simulink model "planta_rots"  (R2025b)
settings: Solver=VariableStepAuto  StartTime=0.0  StopTime=1000  RelTol=1e-3
values from neighbouring files (symbols this model uses):
  ah_max = 0.75    [init_plant_parameters.m]
  at_max = 0.80    (= 0.8)    [init_plant_parameters.m]
  bcx = 1.0e6    (= 1000000)    [init_plant_parameters.m]
  bcy = 10.0e6    (= 10000000)    [init_plant_parameters.m]
  bh_eq = bhm+bhd/ih^2    (= 18.0165289256)    [init_plant_parameters.m]
  bhb = 100e6    (= 100000000)    [init_plant_parameters.m]
  bhEb = 2.2e9    (= 2200000000)    [init_plant_parameters.m]
  bhwu = 150    [init_plant_parameters.m]
  bt = 90.0    (= 90)    [init_plant_parameters.m]
  bt_eq = btm+btd/it^2    (= 6.002)    [init_plant_parameters.m]
  btb = 5.0e6    (= 5000000)    [init_plant_parameters.m]
  btw = 3.0e3    (= 3000)    [init_plant_parameters.m]
  counter_limit = timeout/(Ts0*1000)    (= 1500)    [init_plant_parameters.m]
  envolvent = [ones(1,N_xt)]*38    [init_plant_parameters.m]
  g = 9.80665    [init_plant_parameters.m]
  Hc = 2.59    [init_plant_parameters.m]
  ih = 22.0    (= 22)    [init_plant_parameters.m]
  it = 30.0    (= 30)    [init_plant_parameters.m]
  Jh_eq = Jhm_hb+Jhd_hEb/ih^2    (= 37.8512396694)    [init_plant_parameters.m]
  Jt_eq = Jtm_tb+Jtd/it^2    (= 8.33333333333)    [init_plant_parameters.m]
  k_i_c = abs(polos_obs_c)^3    [init_plant_parameters.m]
  k_i_h = abs(polos_obs_h)^3    [init_plant_parameters.m]
  k_omega_c = 3 * abs(polos_obs_c)^2    [init_plant_parameters.m]
  k_omega_h = 3 * abs(polos_obs_h)^2-k_tita_h*bh_eq/Jh_eq    [init_plant_parameters.m]
  k_tita_c = 3 * abs(polos_obs_c)    [init_plant_parameters.m]
  k_tita_h = 3 * abs(polos_obs_h)-bh_eq/Jh_eq    [init_plant_parameters.m]
  Kcy = 1.8e9    (= 1800000000)    [init_plant_parameters.m]
  khwu = 236e6    (= 236000000)    [init_plant_parameters.m]
  Ki_c = (wn_t^2*Mt)/Kf    (= 320)    [init_plant_parameters.m]
  Ki_i = (wn_h^2)*Jh_eq    (= 2422.47933884)    [init_plant_parameters.m]
  Kp_c = (2*zitta_t*wn_t*Mt)/Kf    (= 1120)    [init_plant_parameters.m]
  Kp_i = 2*zitta_h*wn_h*Jh_eq    (= 1211.23966942)    [init_plant_parameters.m]
  Ktw = 480e3    (= 480000)    [init_plant_parameters.m]
  Lh0 = 110    [init_plant_parameters.m]
  lh_0 = Yt0-yh_0    (= 7)    [init_plant_parameters.m]
  Mc_max = 50000    [init_plant_parameters.m]
  Mc_min = 2000    [init_plant_parameters.m]
  Ms = 15000    [init_plant_parameters.m]
  Mt = 30000    [init_plant_parameters.m]
  P_nom = 956150    [init_plant_parameters.m]
  periodo_pulsos = 100    [init_plant_parameters.m]
  rhd = 0.75    [init_plant_parameters.m]
  rtd = 0.50    (= 0.5)    [init_plant_parameters.m]
  tau_hm = Ts2    (= 0.001)    [init_plant_parameters.m]
  tau_tm = Ts2    (= 0.001)    [init_plant_parameters.m]
  Thb_Max = 50e3    (= 50000)    [init_plant_parameters.m]
  ThEb_Max = 1.1e6    (= 1100000)    [init_plant_parameters.m]
  Thm_0 = 0    [init_plant_parameters.m]
  Thm_Max = 20e3    (= 20000)    [init_plant_parameters.m]
  titahm_0 = yl_0/(rhd/(2*ih))    (= 2228.19975108)    [init_plant_parameters.m]
  titatm_0 = xtd_0/(rtd/it)    (= 300)    [init_plant_parameters.m]
  Ts0 = 0.02    [init_plant_parameters.m]
  Ts1 = 0.02    [init_plant_parameters.m]
  Ts2 = 0.001    [init_plant_parameters.m]
  Ttb_Max = 5.0e3    (= 5000)    [init_plant_parameters.m]
  Ttm_0 = 0    [init_plant_parameters.m]
  Ttm_Max = 4.0e3    (= 4000)    [init_plant_parameters.m]
  vh_0 = 0    [init_plant_parameters.m]
  vh_max = 3    [init_plant_parameters.m]
  vh_nom = 1.5    [init_plant_parameters.m]
  vt_0 = 0    [init_plant_parameters.m]
  vt_max = 4.0    (= 4)    [init_plant_parameters.m]
  Wc = 2.44    [init_plant_parameters.m]
  x_LIDAR = 3    [init_plant_parameters.m]
  xl_0 = 5    [init_plant_parameters.m]
  xt_0 = 5    [init_plant_parameters.m]
  xt_max = 50.0    (= 50)    [init_plant_parameters.m]
  xt_min = -30.0    (= -30)    [init_plant_parameters.m]
  xtd_0 = xt_0    (= 5)    [init_plant_parameters.m]
  yc0_vec_inicial = [ 0, 0, 1, 0, 0, 1, 0, 0, 0, 0, 0, 0, alt_borde,                   3, 5, 6, 3, 5, 6, 6, 4, 1, 1, -4, -5, -2, -1, 2, 6, 4, 2, 5,                   alt_borde] * Hc    [init_plant_parameters.m]
  yh_max = 40    [init_plant_parameters.m]
  yh_min = -20    [init_plant_parameters.m]
  yl_0 = Yt0 - l_0    (= 37.9806775752)    [init_plant_parameters.m]
  Yt0 = 45.0    (= 45)    [init_plant_parameters.m]
  zitta = 0.5    [init_plant_parameters.m]
undefined symbols (not defined in the file or in its folder): DiscIntNeverNeededParam
libraries: dspnetwork x2, sl3dlib x1, simulink_extras x1, hostiolib x1
(part 2 of 2)

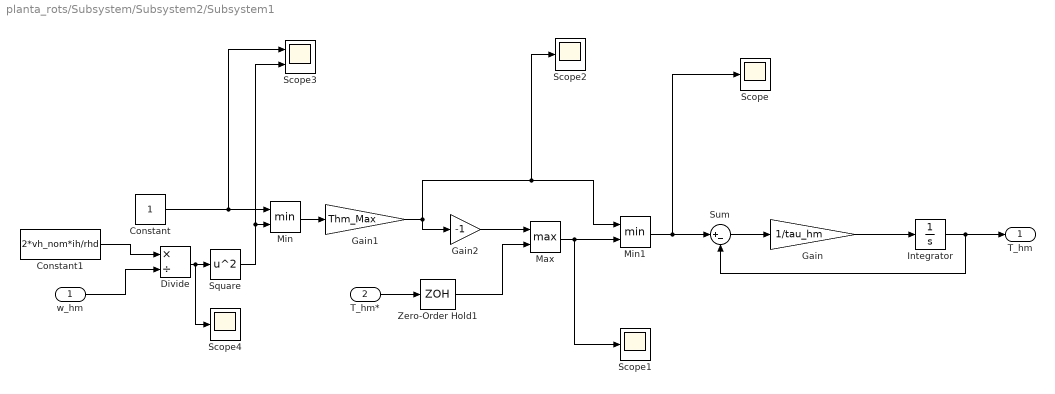
== system planta_rots/Subsystem/Subsystem2/Subsystem1 ==
  w_hm : Inport
  T_hm* : Inport  Port=2
  Constant : Constant
  Constant1 : Constant  Value=2*vh_nom*ih/rhd
  Divide : Product  Inputs=*/
  Gain : Gain  Gain=1/tau_hm
  Gain1 : Gain  Gain=Thm_Max
  Gain2 : Gain  Gain=-1
  Integrator : Integrator
  Max : MinMax  Function=max  Inputs=2
  Min : MinMax  Inputs=2
  Min1 : MinMax  Inputs=2
  Scope{,1..2,4} (4 alike) : Scope
      Scope settings: ActiveDisplayYMinimum=-2500  ActiveDisplayYMaximum=22500  DataLoggingVariableName=ScopeData3
      Scope1 settings: ActiveDisplayYMinimum=-2500  ActiveDisplayYMaximum=22500  DataLoggingVariableName=ScopeData4
      Scope2 settings: ActiveDisplayYMinimum=481.45655  ActiveDisplayYMaximum=22168.72705  DataLoggingVariableName=ScopeData5
      Scope4 settings: ActiveDisplayYMinimum=-0.06596  ActiveDisplayYMaximum=-0.00953  DataLoggingVariableName=ScopeData7
  Scope3 : Scope  NumInputPorts=2
      settings: ActiveDisplayYMinimum=-9.1717430786370772E+28  ActiveDisplayYMaximum=8.25456877077337E+29  DataLoggingVariableName=ScopeData6
  Square : Math  Operator=square
  Sum : Sum  Inputs=|+-
  Zero-Order Hold1 : ZeroOrderHold  SampleTime=tau_hm
  T_hm : Outport
  wires:
  Sum/1 -> Gain/1
  Gain/1 -> Integrator/1
  Integrator/1 -> Sum/2, T_hm/1
  Constant/1 -> Scope3/1, Min/1
  w_hm/1 -> Divide/2
  Constant1/1 -> Divide/1
  Divide/1 -> Scope4/1, Square/1
  Square/1 -> Scope3/2, Min/2
  Min/1 -> Gain1/1
  Gain1/1 -> Scope2/1, Min1/1, Gain2/1
  T_hm*/1 -> Zero-Order Hold1/1
  Gain2/1 -> Max/1
  Max/1 -> Scope1/1, Min1/2
  Min1/1 -> Scope/1, Sum/1
  Zero-Order Hold1/1 -> Max/2

== system planta_rots/Subsystem/accionamiento izaje/brake izaje ==
  w_hm : Inport
  BRK_h : Inport  Port=2
  Constant : Constant  Value=0
  Gain : Gain  Gain=bhb
  Gain1 : Gain  Gain=-Thb_Max
  Switch : Switch  Criteria=u2 > Threshold  SaturateOnIntegerOverflow=off  InputSameDT=off
  Tanh : Trigonometry  Operator=tanh
  T_hb : Outport
  wires:
  Switch/1 -> T_hb/1
  Constant/1 -> Switch/1
  BRK_h/1 -> Switch/2
  w_hm/1 -> Gain/1
  Gain/1 -> Tanh/1
  Tanh/1 -> Gain1/1
  Gain1/1 -> Switch/3

== system planta_rots/Subsystem/accionamiento izaje/brake izaje emergencia ==
  w_hd : Inport
  BRK_hE : Inport  Port=2
  Constant : Constant  Value=0
  Gain : Gain  Gain=bhEb
  Gain1 : Gain  Gain=-ThEb_Max
  Switch : Switch  Criteria=u2 > Threshold  SaturateOnIntegerOverflow=off  InputSameDT=off
  Tanh : Trigonometry  Operator=tanh
  T_hEb : Outport
  wires:
  Tanh/1 -> Gain1/1
  Gain/1 -> Tanh/1
  Constant/1 -> Switch/1
  w_hd/1 -> Gain/1
  Switch/1 -> T_hEb/1
  BRK_hE/1 -> Switch/2
  Gain1/1 -> Switch/3

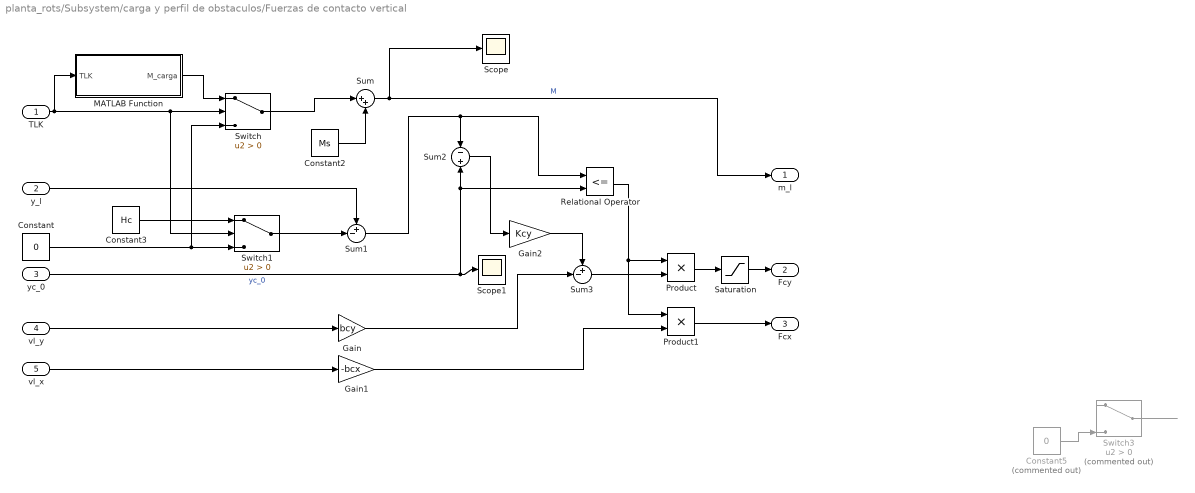
== system planta_rots/Subsystem/carga y perfil de obstaculos/Fuerzas de contacto vertical ==
  TLK : Inport
  y_l : Inport  Port=2
  yc_0 : Inport  Port=3
  vl_y : Inport  Port=4
  vl_x : Inport  Port=5
  Constant : Constant  Value=0
  Constant2 : Constant  Value=Ms
  Constant3 : Constant  Value=Hc
  Constant5 : Constant  Commented=on  Value=0
  Gain : Gain  Gain=bcy
  Gain1 : Gain  Gain=-bcx
  Gain2 : Gain  Gain=Kcy
  MATLAB Function : MATLAB Function  TreatAsAtomicUnit=on
  Product : Product
  Product1 : Product
  Relational Operator : RelationalOperator  Operator=<=  OutDataTypeStr=boolean  RndMeth=Simplest  InputSameDT=off
  Saturation : Saturate  UpperLimit=inf  LowerLimit=0
  Scope : Scope
      settings: ActiveDisplayYMinimum=-30040.049311756404  ActiveDisplayYMaximum=65258.780060315854  DataLoggingVariableName=ScopeData31
  Scope1 : Scope
      settings: ActiveDisplayYMinimum=12.776564460216019  ActiveDisplayYMaximum=15.5369149188378  DataLoggingVariableName=ScopeData32
  Sum : Sum  Inputs=|++
  Sum1 : Sum  Inputs=+-|
  Sum2 : Sum  Inputs=-|+
  Sum3 : Sum  Inputs=+-|
  Switch : Switch  Criteria=u2 > Threshold  SaturateOnIntegerOverflow=off  InputSameDT=off
  Switch1 : Switch  Criteria=u2 > Threshold  SaturateOnIntegerOverflow=off  InputSameDT=off
  Switch3 : Switch  Commented=on  Criteria=u2 > Threshold  SaturateOnIntegerOverflow=off  InputSameDT=off
  m_l : Outport
  Fcy : Outport  Port=2
  Fcx : Outport  Port=3
  wires:
  MATLAB Function/1(M_carga) -> Switch/1
  TLK/1 -> MATLAB Function/1(TLK), Switch1/2, Switch/2
  Constant/1 -> Switch1/3, Switch/3
  Constant3/1 -> Switch1/1
  Switch/1 -> Sum/1
  Sum/1 -> Scope/1, m_l/1  "M"
  Constant2/1 -> Sum/2
  Switch1/1 -> Sum1/2
  y_l/1 -> Sum1/1
  Sum1/1 -> Relational Operator/1, Sum2/1
  yc_0/1 -> Scope1/1, Sum2/2, Relational Operator/2  "yc_0"
  Sum2/1 -> Gain2/1
  Gain2/1 -> Sum3/1
  Relational Operator/1 -> Product1/1, Product/1
  Product1/1 -> Fcx/1
  Gain/1 -> Sum3/2
  vl_y/1 -> Gain/1
  vl_x/1 -> Gain1/1
  Gain1/1 -> Product1/2
  Sum3/1 -> Product/2
  Constant5/1 -> Switch3/3
  Switch3/1 -> ?
  ? -> Switch3/1, Switch3/2
  Product/1 -> Saturation/1
  Saturation/1 -> Fcy/1

== matlab function planta_rots/Subsystem/carga y perfil de obstaculos/MATLAB Function ==
  data: y0_array input; yc0_xt output; index input
function yc0_xt= calcula_y0(y0_array,index)
index = floor(index)+1;
index = min(max(index,1),33);
yc0_xt = y0_array(index);

== stateflow chart planta_rots/Nivel 0 ==
  state Muerto
    entry:
    BRK_hE_N0 = 0; BRK_t_N0 = 0;
  state Name
    state ESTADOS_SEGURIDAD [parallel]
      entry:
      vh_lim = vh_max;
      settings: executionOrder=1
      state SISTEMA_OK
        entry:
        BRK_hE_N0 = 1; BRK_t_N0 = 1;
        FALLA_MAN = 0; FALLA_WD = 0;
        FALLA_IZAJE_SUP = 0; FALLA_IZAJE_INF = 0;
        FALLA_IZAJE_SV = 0;
        FALLA_CARRO_DER = 0; FALLA_CARRO_IZQ = 0;
        during:
        vh_lim = min(vh_max,...
        max(vh_nom, (P_nom / ((m_cont + Ms) * g))));
      state MODO_RECUPERACION
        entry:
        BRK_hE_N0 = 1; BRK_t_N0 = 1;
        FALLA_MAN = 0;
        FALLA_IZAJE_SV = 0;
      state EMERGENCIA_MANUAL
        entry:
        BRK_hE_N0 = 0; BRK_t_N0 = 0;
        FALLA_MAN = 1;
      state EMERGENCIA_IZAJE_INF
        entry:
        BRK_hE_N0 = 0; BRK_t_N0 = 1;
        FALLA_IZAJE_INF = 1;
      state EMERGENCIA_IZAJE_SUP
        entry:
        BRK_hE_N0 = 0; BRK_t_N0 = 1;
        FALLA_IZAJE_SUP = 1;
      state EMERGENCIA_CARRO_SV
        entry:
        BRK_hE_N0 = 1; BRK_t_N0 = 0;
        FALLA_CARRO_SV = 1;
      state EMERGENCIA_CARRO_DER
        entry:
        BRK_hE_N0 = 1; BRK_t_N0 = 0;
        FALLA_CARRO_DER = 1;
      state EMERGENCIA_CARRO_IZQ
        entry:
        BRK_hE_N0 = 1; BRK_t_N0 = 0;
        FALLA_CARRO_IZQ = 1;
      state EMERGENCIA_IZAJE_SV
        entry:
        BRK_hE_N0 = 0; BRK_t_N0 = 1;
        FALLA_IZAJE_SV = 1;
      (default) -> SISTEMA_OK
      MODO_RECUPERACION -> SISTEMA_OK : [recup_ok == 1]
      (junction 76) -> MODO_RECUPERACION : [BTN_Reset]
      SISTEMA_OK -> (junction 55) [order 3]
      SISTEMA_OK -> (junction 48) [order 2]
      SISTEMA_OK -> EMERGENCIA_MANUAL [order 1] : [BTN_Emerg]
      EMERGENCIA_MANUAL -> (junction 76)
      (junction 78) -> (junction 76)
      (junction 55) -> EMERGENCIA_IZAJE_SV [order 3] : [abs(vh_obs) > (1.15 * vh_lim)]
      (junction 55) -> EMERGENCIA_CARRO_SV [order 4] : [abs(vt_obs) > (1.15 * vt_max)]
      (junction 48) -> EMERGENCIA_CARRO_DER [order 2] : [FCE_der == 1]
      (junction 48) -> EMERGENCIA_CARRO_IZQ [order 1] : [FCE_izq == 1]
      (junction 55) -> EMERGENCIA_IZAJE_INF [order 2] : [FCE_inf == 1]
      (junction 55) -> EMERGENCIA_IZAJE_SUP [order 1] : [FCE_sup == 1]
      EMERGENCIA_CARRO_DER -> (junction 84)
      EMERGENCIA_CARRO_IZQ -> (junction 84)
      EMERGENCIA_IZAJE_INF -> (junction 84)
      EMERGENCIA_IZAJE_SUP -> (junction 78)
      EMERGENCIA_CARRO_SV -> (junction 78)
      EMERGENCIA_IZAJE_SV -> (junction 78)
      (junction 84) -> (junction 78)
    state WATCHDOG [parallel]
      settings: executionOrder=2
      state HEARTBEAT_DOWN
        entry:
        WD_counter = 0;
        during:
        WD_counter = WD_counter + 1;
      state DETECCION_FALLO
        entry:
        FALLA_WD = 1;
      state HEARTBEAT_UP
        entry:
        WD_counter = 0;
        during:
        WD_counter = WD_counter + 1;
      (default) -> HEARTBEAT_DOWN
      HEARTBEAT_DOWN -> DETECCION_FALLO [order 2] : [WD_counter >= counter_limit]
      HEARTBEAT_UP -> HEARTBEAT_DOWN [order 1] : [heartbeat==0]
      HEARTBEAT_DOWN -> HEARTBEAT_UP [order 1] : [heartbeat==1]
      DETECCION_FALLO -> HEARTBEAT_DOWN : [FALLA_WD==0]
      HEARTBEAT_UP -> DETECCION_FALLO [order 2] : [WD_counter >= counter_limit]
  (default) -> Muerto
  Muerto -> Name : [modo_muerto==0]
  Name -> Muerto : [modo_muerto==1]
  data: BTN_Emerg input; BTN_Reset input; FCE_der input; FCE_inf input; FCE_izq input; FCE_sup input; P_nom parameter; g parameter; recup_ok input; vh_max parameter; vh_nom parameter; vh_obs input; vh_lim local; BRK_hE_N0 output; BRK_t_N0 output; FALLA_CARRO_DER output; FALLA_CARRO_IZQ output; FALLA_IZAJE_INF output; FALLA_IZAJE_SUP output; FALLA_IZAJE_SV output; FALLA_MAN output; FALLA_WD output; vt_max parameter; vt_obs input; FALLA_CARRO_SV output; modo_muerto input; counter_limit parameter; heartbeat input; WD_counter local; Ms parameter; m_cont input

== stateflow chart planta_rots/Nivel 1 ==
  state Muerto
    entry:
    modo_muerto=1;
    BRK_h_N1=0;
    BRK_t_N1=0;
    modo_reposo =0;
    TLK = 0;
    exit:
    modo_muerto=0;
  state Automata
    state AUTOMATA_PRINCIPAL [parallel]
      entry:
      ya_vuelvo = 0;
      dead_zone = 0.1; % Zona muerta joystick
      %error_der = 0; error_izq = 0;
      %error_sup = 0; error_inf = 0;
      %error_otro =1;
      %modo_manual_auto = 0;
      %ya_vuelvo = 0;
      during:
      Joy_CMD_X = Joy_XY(1);
      Joy_CMD_Y = Joy_XY(2);
      settings: executionOrder=6
      state REPOSO
        entry:
        modo_reposo = 1;
        BRK_t_N1 = 0; BRK_h_N1 = 0;
        modo_manual = 0;
        modo_manual_auto =0;
        error_der = 0; error_izq = 0;
        error_sup = 0; error_inf = 0;
        error_otro =0;
        modo_error = 0;
        exit:
        modo_reposo = 0;
      state RECUPERACION
        entry:
        BRK_t_N1 = 1; BRK_h_N1 = 1;
        vel_error = 0.1;
        recuperacion = 1;
        during:
        if (abs(Joy_CMD_X) < dead_zone)
        vx_target = 0;
        else
        vx_target = Joy_CMD_X * vt_max/3;
        if (error_der == 1)
        vx_target = Joy_CMD_X * vel_error;
        if (vx_target > 0) vx_target = 0; end
        elseif (error_izq == 1)
        vx_target = Joy_CMD_X * vel_error;
        if (vx_target < 0) vx_target = 0; end
        end
        end
        if (abs(Joy_CMD_Y) < dead_zone)
        vy_target = 0;
        else
        vy_target = Joy_CMD_Y * vh_lim/3;
        if (error_sup == 1)
        vy_target = Joy_CMD_Y * vel_error;
        if (vy_target > 0) vy_target = 0; end
        elseif (error_inf == 1)
        vy_target = Joy_CMD_Y * vel_error;
        if (vy_target < 0) vy_target = 0; end
        end
        end
        exit:
        recuperacion = 0;
        %modo_error = 1;
      state ERROR_OTRO
        entry:
        BRK_t_N1 = 0; BRK_h_N1 = 0;
        recuperacion = 0;
        error_otro = 1;
        vx_target=0,vy_target=0;
        modo_error = 1;
      state ERROR_FC_sup_inf
        entry:
        BRK_t_N1 = 1; BRK_h_N1 = 0;
        vy_target = 0;
        recuperacion = 0;
        if FC_inf==1
        error_inf=1;
        elseif FC_sup==1;
        error_sup=1;
        end
        modo_error = 1;
      state MANUAL
        entry:
        %BRK_t_N1 = 1; BRK_h_N1 = 1;
        modo_manual = 1;
        during:
        if (abs(T_hm)>(m_container+Ms)*g*0.02)
        BRK_h_N1=1;
        end
        if (abs(T_tm)>(m_container+Ms)*g*0.0002)
        BRK_t_N1=1;
        end
        if (abs(Joy_CMD_X) < dead_zone)
        vx_target = 0;
        else
        vx_target = Joy_CMD_X * vt_max;
        end
        if (abs(Joy_CMD_Y) < dead_zone)
        vy_target = 0;
        else
        vy_target = Joy_CMD_Y * vh_lim;
        end
        exit:
        modo_manual = 0;
      state ERROR_FC_izq_der
        entry:
        BRK_t_N1 = 0; BRK_h_N1 = 1;
        vx_target = 0;
        recuperacion = 0;
        if FC_der==1;
        error_der=1;
        elseif FC_izq==1;
        error_izq=1;
        end
        modo_error = 1;
      state MODO_AUTO
        entry:
        if(ya_vuelvo == 1)
        BRK_t_N1 = 1; BRK_h_N1 = 1;
        else ya_vuelvo = 0;
        end
        ciclo_doble=0;
        ejec_mov_final = 0;
        exit:
        if(ya_vuelvo == 0)
        modo_auto = 0;
        modo_manual_auto = 0;
        ejec_mov = 0;
        end
        state SEL_ORIGEN
          entry:
          i_sel = 1;
          i_origen = 0;
          cont =0;
          during:
          if (Joy_CMD_X > dead_zone) && every(50, tick)
          i_sel = i_sel + 1;
          elseif (Joy_CMD_X < -dead_zone) && every(50, tick)
          i_sel = i_sel - 1;
          end
          cont= Check_Container(i_sel,yc0_vec);
          exit:
          i_origen = i_sel;
        state SEL_DESTINO
          entry:
          i_sel = i_origen;
          i_destino = 0;
          invalido = 1;
          during:
          if (Joy_CMD_X > dead_zone) && every(50, tick)
          i_sel = i_sel + 1;
          elseif (Joy_CMD_X < -dead_zone) && every(50, tick)
          i_sel = i_sel - 1;
          end
          if (i_sel == 33 || i_sel == 13 || i_sel == 1|| i_sel==i_origen)
          invalido = 1;
          else invalido = 0;
          end
          exit:
          i_destino = i_sel;
        state AUTO_INIT
          entry:
          BRK_t_N1 = 0; BRK_h_N1 = 0;
          home = 13;
          estado = 1; % Etapa de movimiento
          if (TLK == 1)
          estado = 2;
          i_origen = 0;
          end
        state SELECCION_TRAYECTORIA
          entry:
          modo_auto = 1;
          manual_ok = 0;
          i_usado = 1;
          if (estado == 1)
          i_usado = i_origen;
          elseif (estado == 2)
          i_usado = i_destino;
          elseif (estado ==3);
          i_usado = home;
          end
        state MOVIMIENTO_CURVO
          entry: ejec_mov = 1;ya_vuelvo=0;
          during:
          if (abs(T_hm)>(m_container+Ms)*g*0.02)
          BRK_h_N1=1;
          end
          if (abs(T_tm)>(m_container+Ms)*g*0.0002)
          BRK_t_N1=1;
          end
          [vx_target, vy_target, manual_ok] = Planificador_Trayectoria_Vel(xt_enc,...
          yh_enc, vt_obs, vh_obs, i_usado, envolvente, TLK, theta_l, vh_lim);
          if (abs(Joy_XY(1)) > dead_zone || abs(Joy_XY(2)) > dead_zone)
          ya_vuelvo = 1
          end
          if (BTN_Auto ==1)
          ciclo_doble=1;
          end
          exit: ejec_mov = 0;
        state MOVIMIENTO_CURVO_FINAL
          entry: ejec_mov_final = 1;ya_vuelvo=0;
          during:
          if (abs(T_hm)>(m_container+Ms)*g*0.02)
          BRK_h_N1=1;
          end
          if (abs(T_tm)>(m_container+Ms)*g*0.0002)
          BRK_t_N1=1;
          end
          [vx_target, vy_target, manual_ok] = Planificador_Trayectoria_Vel(xt_enc,...
          yh_enc, vt_obs, vh_obs, i_usado, envolvent, TLK, theta_l, vh_lim);
          if (abs(Joy_XY(1)) > dead_zone || abs(Joy_XY(2)) > dead_zone)
          ya_vuelvo = 1
          end
          exit: ejec_mov_final = 0;
        state MODO_MANUAL_SIMPLE
          entry:
          modo_auto = 0;
          modo_manual_auto = 1;
          during:
          if (abs(T_hm)>(m_container+Ms)*g*0.02)
          BRK_h_N1=1;
          end
          if (abs(T_tm)>(m_container+Ms)*g*0.0002)
          BRK_t_N1=1;
          end
          if (abs(Joy_CMD_X) < dead_zone)
          vx_target = 0;
          else
          vx_target = Joy_CMD_X * 0.05;
          end
          if (abs(Joy_CMD_Y) < dead_zone)
          vy_target = 0;
          else
          vy_target = Joy_CMD_Y * vh_lim;
          end
          exit:
          estado = estado + 1;
          modo_manual_auto = 0;
        (default) -> (junction 347)
        (junction 347) -> MOVIMIENTO_CURVO [order 1] : [ya_vuelvo == 1]
        (junction 347) -> AUTO_INIT [order 2]
        SEL_ORIGEN -> SEL_DESTINO : [BTN_TLK &&...
            |  cont == 1]
        MODO_MANUAL_SIMPLE -> AUTO_INIT [order 1] : [TLK == 0 && yh_enc > (envolvente(i_usado) + Hc) &&...
            |  abs(vh_obs) < 0.1 && estado == 2 && ciclo_doble ==1]
        AUTO_INIT -> (junction 245)
        (junction 245) -> SEL_ORIGEN [order 2] : [TLK == 0]
        (junction 245) -> SEL_DESTINO [order 1] : [TLK == 1]
        SEL_DESTINO -> SELECCION_TRAYECTORIA : [BTN_TLK &&...
            |  invalido == 0]
        SELECCION_TRAYECTORIA -> MOVIMIENTO_CURVO_FINAL [order 1] : [estado == 3]
        SELECCION_TRAYECTORIA -> MOVIMIENTO_CURVO [order 2]
        MODO_MANUAL_SIMPLE -> SELECCION_TRAYECTORIA [order 2] : [(TLK == 1 && yh_enc > (envolvente(i_usado) + Hc) &&...
            |  abs(vh_obs) < 0.1 && estado == 1) ||...
            | (TLK == 0 && yh_enc > (envolvente(i_usado) + Hc) &&...
            |  abs(vh_obs) < 0.1 && estado == 2)]
        MOVIMIENTO_CURVO -> MODO_MANUAL_SIMPLE [order 1] : [manual_ok == 1]
      (default) -> REPOSO
      RECUPERACION -> REPOSO [order 1] : [(yh_enc < yh_max*0.99) &&...
          |  (yh_enc > yh_min*0.99) &&...
          |  (xt_enc < xt_max*0.99) &&...
          |  (xt_enc > xt_min*0.99)]
      MODO_AUTO -> REPOSO [order 2] : [ejec_mov_final == 1 &&...
          |  (sobrecarga==1 || (TLK == 0 &&...
          |  abs(yh_enc - envolvent(i_usado))<0.1 &&...
          |  abs(vh_obs) < 0.1 && estado == 3)&&...
          |  i_carro == i_usado && abs(vt_obs)<0.1)]
      MODO_AUTO -> REPOSO [order 1] : [BTN_Reset == 1]
      REPOSO -> MODO_AUTO [order 2] : [BTN_Auto == 1 && scan==1]
      REPOSO -> MANUAL [order 1] : [abs(Joy_XY(1)) > dead_zone ||...
          |  abs(Joy_XY(2)) > dead_zone]
      MANUAL -> REPOSO [order 2] : [duration((abs(Joy_XY(1)) < 0.1 &&...
          |  abs(Joy_XY(2)) < 0.1 &&...
          |  abs(vt_obs) < 0.01 &&...
          |  abs(vh_obs) < 0.01 &&...
          |  abs(theta_l_dot) < 0.006 &&...
          |  abs(theta_l) < 0.006), sec) > 1]
      ERROR_OTRO -> (junction 167)
      (junction 102) -> ERROR_OTRO [order 3] : [(FALLA_MAN == 1 ||...
          |  FALLA_WD == 1 ||...
          |  FALLA_SV ==1) &&...
          |  error_otro == 0]
      (junction 102) -> ERROR_FC_sup_inf [order 1] : [(FC_inf == 1&&...
          | error_inf==0) ||...
          | (FC_sup == 1&&...
          | error_sup==0)]
      ERROR_FC_sup_inf -> (junction 167)
      (junction 167) -> RECUPERACION : [BTN_Reset==1]
      ERROR_FC_izq_der -> (junction 167)
      (junction 102) -> ERROR_FC_izq_der [order 2] : [(FC_izq == 1&&...
          | error_izq==0)||...
          | (FC_der == 1&&...
          | error_der==0)]
      RECUPERACION -> (junction 102) [order 2]
      MANUAL -> (junction 102) [order 1]
      MODO_AUTO -> (junction 102) [order 3]
      MOVIMIENTO_CURVO -> MANUAL [order 2] : [ya_vuelvo==1]
    state TWISTLOCKS [parallel]
      entry:
      m_container=0;
      settings: executionOrder=1
      state VACIO
        entry:
        TLK = 0;
        m_est = Ms;
        sobrecarga = 0;
        during:
        hay_cont = Check_Container...
        (i_carro, yc0_vec);
        vh_lim = vh_max;
      state CERRANDO_TLK
        entry:
        TLK = 1;
        y_start = yh_enc;
        during:
        vh_lim = 0.1;
        vx_target = 0;
        % Filtro
        m_est = m_est + 0.1 *...
        (max(Ms, (Fhw * 2 / g)) - m_est);
        m_container=m_est-Ms;
      state CARGADO
        entry:
        m_container = m_est - Ms; % Masa estimada container
        if (m_container > (Mc_max + 100)) % Margen de 100kg
        sobrecarga = 1;
        end
        during:
        %m_est = max(Ms, (Fhw * 2 / g));
        vh_lim = min(vh_max,...
        max(vh_nom, P_nom / ((m_container + Ms) * g)));
        if (sobrecarga == 1)
        vh_lim = 0.1; vx_target = 0;
        if (vy_target > 0) vy_target = 0; end
        end
      state ABRIENDO_TLK
        entry:
        TLK = 0;
        y_start = yh_enc;
        m_container = 0;
        sobrecarga = 0;
        during:
        m_est = max(Ms, Fhw * 2 / g);
        vh_lim = 0.1;
        vx_target = 0;
      (default) -> VACIO
      VACIO -> CERRANDO_TLK : [(BTN_TLK == 1) &&...
          |  Fhw < (Ms*g/2 * 0.8) &&...
          |  hay_cont == 1]
      ABRIENDO_TLK -> VACIO : [Fhw > (Ms*g/2*0.8) &&...
          |  abs(yh_enc - y_start) > 0.3 &&...
          |  abs(vt_obs) < 0.01]
      CERRANDO_TLK -> CARGADO : [Fhw > (Ms*g/2 * 1.2) &&...
          |  abs(yh_enc - y_start) > 0.3 &&...
          |  abs(vt_obs) < 0.01]
      CARGADO -> ABRIENDO_TLK : [(BTN_TLK == 1) &&...
          |  Fhw < ((m_est*g/2)*0.8) &&...
          | ~ismember(i_carro, [1, 13, 33])]
    state INDICES_PERFIL [parallel]
      settings: executionOrder=2
      state Escaneo [parallel]
        entry:
        scan=1;
        flag1 =0;
        flag2=0;
        during:
        if i_lidar ==33
        flag1 = 1;
        end
        if i_lidar==2
        flag2 = 1;
        end
        if flag1 == 1 && flag2 ==1
        scan=1;
        end
        settings: executionOrder=3
      state INDICES [parallel]
        entry:
        i_carro = 1; i_lidar = 4;
        during:
        i_carro = floor((xt_enc - xt_min)/Wc) + 1;
        i_lidar = floor((xt_enc+x_LIDAR-xt_min)/Wc)+1;
        i_carro = min(max(i_carro,1),33);
        i_lidar = min(max(i_lidar ,1),33);
        settings: executionOrder=1
      state ACTUALIZAR_PERFIL_ALTURAS [parallel]
        entry:
        yc0_vec = yc0_vec_inicial; yc0 = 0;
        TLK_anterior = 0;
        during:
        TLK_rise  = (TLK_anterior == 0) && (TLK == 1);
        TLK_fall  = (TLK_anterior == 1) && (TLK == 0);
        if(TLK_rise) % Si agarré un container, hay que bajar el perfi
        yc0_vec(i_carro) = yc0_vec(i_carro) - Hc;
        elseif(TLK_fall) % Si solté un container, hay que subir el perfil
        yc0_vec(i_carro) = yc0_vec(i_carro) + Hc;
        end
        TLK_anterior = TLK; yc0 = yc0_vec(i_carro);
        envolvente = Generar_Envolvente(yc0_vec);
        settings: executionOrder=2
    state VELOCIDAD_LIMITES [parallel]
      during:
      % LÍMITE INFERIOR DE IZAJE
      if (TLK == 1)
      dist = yh_enc - (yc0 + 0.5 + Hc); T_retardo = 0.8;
      else
      dist = yh_enc - (yc0 + 0.5); T_retardo = 0.4;
      end
      % Compensación con retardo dinámico
      dist_efectiva = dist - (abs(vy_suave) * T_retardo);
      if (dist_efectiva < 0)
      dist_efectiva = 0;
      end
      acc_plan = ah_max * 0.5;
      v_segura = sqrt(0.01 + 2 * acc_plan * dist_efectiva);
      if (v_segura > vh_lim)
      v_segura = vh_lim;
      end
      % Si pide moverse más rápido, se recorta
      if (vy_suave < -v_segura)
      vy_suave = -v_segura;
      end
      % LÍMITE SUPERIOR DE IZAJE
      dist = (yh_max - 2) - yh_enc;
      dist_efectiva = dist - (abs(vy_suave) * T_retardo);
      if (dist_efectiva < 0)
      dist_efectiva = 0;
      end
      v_segura = sqrt(0.01 + 2 * acc_plan * dist_efectiva);
      if (v_segura > vh_lim)
      v_segura = vh_lim;
      end
      if (vy_suave > v_segura)
      vy_suave = v_segura;
      end
      % LÍMITE DERECHO DEL CARRO
      T_retardo = 5; % Retardo mayor para el carro
      dist = (xt_max - 2) - xt_enc;
      dist_efectiva = dist - (abs(vx_suave) * T_retardo);
      if (dist_efectiva < 0)
      dist_efectiva = 0;
      end
      acc_plan = at_max * 0.5;
      v_segura = sqrt(0.01 + 2 * acc_plan * dist_efectiva);
      if (vx_suave > v_segura)
      vx_suave = v_segura;
      end
      % LÍMITE IZQUIERDO DEL CARRO
      dist = xt_enc - (xt_min + 2);
      dist_efectiva = dist - (abs(vx_suave) * T_retardo);
      if (dist_efectiva < 0)
      dist_efectiva = 0;
      end
      v_segura = sqrt(0.01 + 2 * acc_plan * dist_efectiva);
      if (vx_suave < -v_segura)
      vx_suave = -v_segura;
      end
      settings: executionOrder=3
    state SUAVIZADO_VELOCIDAD [parallel]
      entry:
      ax_act = 0; ay_act = 0;
      jerk_max = 1.5;
      vx_suave = 0; vy_suave = 0;
      vx_target = 0; vy_target = 0;
      during:
      [vx_suave, ax_act] = Suavizador_Cinematico...
      (vx_target, vx_suave, ax_act, at_max, jerk_max);
      [vy_suave, ay_act] = Suavizador_Cinematico...
      (vy_target, vy_suave, ay_act, ah_max, jerk_max);
      settings: executionOrder=4
    state WATCHDOG_HEARTBEAT [parallel]
      settings: executionOrder=5
      state PULSOS_UP
        entry:
        heartbeat = 0;
      state PULSOS_DOWN
        entry:
        heartbeat = 1;
      (default) -> PULSOS_UP
      PULSOS_DOWN -> PULSOS_UP : [after(periodo_pulsos, msec)]
      PULSOS_UP -> PULSOS_DOWN : [after(periodo_pulsos, msec)]
  (default) -> Muerto
  Muerto -> Automata : [BTN_ON_OFF==1]
  Automata -> Muerto : [duration((BTN_ON_OFF==0 && modo_reposo == 1),sec)>2 && ...
      | duration(TLK==0,sec)>2]
  data: i_pos function_input; y0_vec function_input; hay_container function_output; x_real function_input; y_real function_input; vx_carro function_input; vy_izaje function_input; i_ref function_input; envolvente_vec function_input; twistlock function_input; tita_l function_input; vh_limit function_input; vx_ref function_output; vy_ref function_output; listo function_output; perfil_escaneado_vec function_input; envolvente_f function_output; v_target function_input; v_act function_input; a_act function_input; A_MAX function_input; J_MAX function_input; v_out function_output; a_out function_output; BTN_ON_OFF input; Joy_XY input; theta_l input; theta_l_dot input; vh_obs input; vt_obs input; BRK_h_N1 output size=1; BRK_t_N1 output size=1; Joy_CMD_X local; Joy_CMD_Y local; dead_zone local; Fhw input; yh_enc input; TLK output size=1 =0; hay_cont local; y_start local; BTN_TLK input; Hc parameter; yc0_vec output size=[1 33]; TLK_anterior local; TLK_fall local; TLK_rise local; yc0 local; Ms parameter; g parameter; Mc_max parameter; Wc parameter; ah_max parameter; at_max parameter; x_LIDAR parameter; xt_max parameter; xt_min parameter; yc0_vec_inicial parameter; yh_max parameter; T_retardo local; acc_plan local; dist local; dist_efectiva local; v_segura local; i_lidar local; xt_enc input; vh_nom parameter; vt_max parameter; P_nom parameter; i_carro local; vh_max parameter; vh_lim local size=1; BTN_Reset input; FC_der input; FC_inf input; FC_izq input; FC_sup input; vel_error local; error_der local; error_inf local; error_izq local; error_sup local; yh_min parameter; i_lista local; BTN_Auto input; i_origen local =1; i_destino local =1; x_origen local =0; x_inicio local =0; debounce local =0; ejec_mov local; invalido local; manual_ok local; i_usado local; estado local; cont local; envolvente local; i_sel output =1; ax_act local; ay_act local; jerk_max local; vx_suave output size=1; vy_suave output size=1; vx_target local size=1; vy_target local size=1; ya_vuelvo local; recuperacion output size=1; FALLA_MAN input; FALLA_WD input; error_otro local; FALLA_SV input; T_hm input; T_tm input; modo_muerto output size=1; periodo_pulsos parameter; heartbeat output size=1; flag1 local; scan local; flag2 local; m_est local size=1; m_container output size=1; home local; envolvent parameter; ejec_mov_final local; ciclo_doble local; modo_auto output =0; modo_manual output size=1; modo_manual_auto output; modo_reposo output =0; modo_error output; sobrecarga output
  function hay_container = Check_Container(...:
    | function hay_container = Check_Container(...
    |     i_pos, y0_vec)
    | 
    | if(i_pos<13 && y0_vec(i_pos)>0)
    |    hay_container = 1;
    | elseif(i_pos>13 && i_pos<33 && y0_vec(i_pos)>-18)
    |    hay_container = 1;
    | else
    |    hay_container = 0;
    | end
    | 
    | end
  function [vx_ref, vy_ref, listo] = Planificador_Trayectoria_Vel(x_real, y_real,...:
    | function [vx_ref, vy_ref, listo] = Planificador_Trayectoria_Vel(x_real, y_real,...
    |     vx_carro, vy_izaje, i_ref, envolvente_vec, twistlock, tita_l, vh_limit)
    | 
    | %% 1. INICIALIZACIÓN
    | persistent last_i_ref
    | if isempty(last_i_ref)
    |     last_i_ref = -1;
    | end
    | if i_ref ~= last_i_ref
    |     last_i_ref = i_ref;
    | end
    | 
    | %% 2. PARÁMETROS GLOBALES FÍSICOS
    | Kp_x = 0.20;  
    | Kd_x = 0.15;
    | Kp_y = 0.38;
    | Kd_y = 0.25;
    | 
    | H_extra = double(twistlock == 1) * Hc;
    | 
    | %% 3. MAPEO DE LA RUTA Y OBSTÁCULOS
    | i_obj = min(max(i_ref, 1), 33);
    | i_act = min(max(floor((x_real - xt_min) / Wc) + 1, 1), 33);
    | x_dest = xt_min + (i_obj - 0.5) * Wc;
    | 
    | step = sign(i_obj - i_act);
    | if step == 0; step = 1; end
    | 
    | h_obst_fwd = 0;
    | for k = i_act : step : i_obj
    |     if envolvente_vec(k) > h_obst_fwd
    |         h_obst_fwd = envolvente_vec(k);
    |     end
    | end
    | y_techo_ruta = h_obst_fwd + H_extra;
    | 
    | %% 4. SINCRONIZACIÓN CINEMÁTICA
    | % Escaneamos las columnas por delante para ver cuánto tiempo necesitamos para subir
    | limite_vx_sinc = vt_max;
    | 
    | for k = i_act : step : i_obj
    |     techo_seguro = envolvente_vec(k) + H_extra;
    |     dy = techo_seguro - y_real;
    |     
    |     if dy > 0  % Si esa columna está más alta que mi posición actual
    |         xc = xt_min + (k - 0.5) * Wc;
    |         
    |         % Distancia horizontal hasta la "pared" de esa celda
    |         dx = abs(xc - x_real) - (Wc / 2); 
    |         dx = max(0.01, dx); % Evitamos división por cero si estamos muy pegados
    |         
    |         % Tiempo que nos tomará subir ese 'dy' yendo a velocidad de izaje
    |         tiempo_para_subir = dy / vh_limit;
    |         
    |         % La velocidad en X permitida para que nos dé el tiempo de subir sin chocar
    |         vx_max_permitida = (dx + 1.5) / tiempo_para_subir;
    |         
    |         % Nos quedamos siempre con el límite más restrictivo de todo el camino
    |         if vx_max_permitida < limite_vx_sinc
    |             limite_vx_sinc = vx_max_permitida;
    |         end
    |     end
    | end
    | 
    | % Mantenemos una velocidad mínima de 0.10 m/s para que nunca se congele
    | limite_vx_final = max(0.10, min(vt_max, limite_vx_sinc));
    | 
    | % Control PD para el carro
    | l = 45 - y_real;  
    | x_carga   = x_real + l * sin(tita_l);
    | e_x   = x_dest - x_carga;
    | vx_req = Kp_x * e_x - Kd_x * vx_carro;
    | 
    | % Saturamos la referencia con nuestro nuevo límite inteligente
    | vx_ref = max(-limite_vx_final, min(limite_vx_final, vx_req));
    | 
    | %% 5. PLANIFICACIÓN VERTICAL EN Y
    | h_dest_final = envolvente_vec(i_obj) + H_extra;
    | 
    | if abs(x_real - x_dest) < (Wc * 0.4)
    |     y_target = h_dest_final;
    | else
    |     y_target = max(h_dest_final, y_techo_ruta + 1);
    | end
    | 
    | % Control PD para el izaje
    | vy_req = Kp_y * (y_target - y_real) - Kd_y * vy_izaje;
    | vy_ref = max(-vh_limit, min(vh_limit, vy_req));
    | 
    | %% 6. SEÑAL DE LISTO
    | listo = double( ...
    |     abs(x_real - x_dest) < 0.05 && ...          
    |     abs(y_real - h_dest_final) < 0.1 && ...     
    |     abs(tita_l) < 0.0174 && ...                 
    |     abs(vx_carro) < 0.05 &&...
    |     abs(vy_izaje) < 0.05);                    
    | end
  function envolvente_f = Generar_Envolvente...:
    | function envolvente_f = Generar_Envolvente...
    |     (perfil_escaneado_vec)
    | 
    | N = 33; % No puedo usar N_xt, da error
    | h_seguridad = Hc/2; % Margen fijo (ajustable)
    | escaneado_vec = ones(N,1);
    | perfil_seguro = zeros(N,1);
    | for i = 1:N
    |     if escaneado_vec(i) == 1
    |         perfil_seguro(i) = perfil_escaneado_vec(i) + h_seguridad;
    |     else
    |         perfil_seguro(i) = 0;
    |     end
    | end
    | 
    | envolvente_f = perfil_seguro;
    | 
    | for i = 1:N
    |     if escaneado_vec(i) == 0
    |         continue;
    |     end
    | 
    |     e_i = perfil_seguro(i);
    |     % vecino izquierdo
    |     if i > 1 && escaneado_vec(i-1) == 1
    |         if e_i > perfil_seguro(i-1)
    |             envolvente_f(i-1) = max(envolvente_f(i-1), e_i);
    |         end
    |     end
    |     % vecino derecho
    |     if i < N && escaneado_vec(i+1) == 1
    |         if e_i > perfil_seguro(i+1)
    |             envolvente_f(i+1) = max(envolvente_f(i+1), e_i);
    |         end
    |     end
    | end
    | 
    | for i = 1:N
    |     if escaneado_vec(i) == 0
    |         envolvente_f(i) = 0;
    |     end
    | end
    | 
    | end
  function [v_out, a_out] = Suavizador_Cinematico...:
    | function [v_out, a_out] = Suavizador_Cinematico...
    |     (v_target, v_act, a_act, A_MAX, J_MAX)
    | 
    | err_v = v_target - v_act;   % Error instantáneo de velocidad    
    | zona_lineal = 0.05;         % Zona lineal cercana a cero para evitar singularidad en la raíz
    | 
    | %% Generación de aceleración deseada
    | if abs(err_v) < 1e-6        % Evita micro-oscilaciones cuando el error es prácticamente cero.
    |     v_out = v_target;
    |     a_out = 0;
    |     return;
    | % Ley tipo raíz cuadrada
    | elseif abs(err_v) > zona_lineal        
    |     a_req = sign(err_v) * sqrt(2 * J_MAX * abs(err_v)); % Región no lineal
    | else
    |     a_req = (err_v / zona_lineal) * sqrt(2 * J_MAX * zona_lineal);  % Región lineal cercana a cero para evitar pendiente infinita
    | end
    | 
    | %% Saturación de aceleración
    | if a_req > A_MAX
    |     a_req = A_MAX;
    | elseif a_req < -A_MAX
    |     a_req = -A_MAX;
    | end
    | 
    | %% Cálculo de jerk requerido
    | jerk_req = (a_req - a_act) / 0.02;
    | % Saturación de jerk
    | if jerk_req > J_MAX
    |     jerk_req = J_MAX;
    | elseif jerk_req < -J_MAX
    |     jerk_req = -J_MAX;
    | end
    | 
    | %% Integración discreta (Euler)
    | a_out = a_act + jerk_req * 0.02;
    | v_out = v_act + a_out * 0.02;
    | 
    | %% Eliminación de deriva
    | % Forzar a cero absoluto si el joystick está suelto
    | if abs(v_target) < 0.001 && abs(v_out) < 0.001
    |     v_out = 0.0;
    |     a_out = 0.0;
    | end
    | 
    | end

== matlab function planta_rots/Subsystem/carga y perfil de obstaculos/Fuerzas de contacto vertical/MATLAB Function ==
  data: TLK input; M_carga output; Mc_min parameter; Mc_max parameter
function M_carga = Masa_Aleatoria(TLK, Mc_min, Mc_max)
    persistent masa_actual;
    persistent ultimo_estado_trigger;
    
    % Inicialización
    if isempty(masa_actual)
        masa_actual = Mc_min; % Empezamos con el valor mínimo por defecto
        ultimo_estado_trigger = 0;
    end
    
    % DETECCIÓN DE FLANCO DE SUBIDA (Rising Edge)
    if (TLK == 1 && ultimo_estado_trigger == 0)
        % Generar carga aleatoria entre 3tn y 55tn (para tener sobrecarga)
        masa_actual = Mc_min + (Mc_max + 5000 - Mc_min) * rand();
        %masa_actual = Mc_max *3;
        masa_actual = round(masa_actual); 
    end
    
    % Actualizar memoria del trigger
    ultimo_estado_trigger = TLK;
    % Salida: La masa se mantiene constante hasta el próximo trigger
    M_carga = masa_actual;
end

== matlab function planta_rots/Control Joystick /MATLAB Function ==
  data: BTN input; BTN_re output
function BTN_re = fcn(BTN)
    persistent prev;
    persistent state;
    if isempty(prev)
        prev = 0;
        state = 0;
    end
    if BTN == 1 && prev == 0
        state = double(~logical(state));
    end
    BTN_re = state;
    prev = double(BTN);
end

== matlab function planta_rots/Nivel 2/MATLAB Function ==
  settings: updateMethod=DISCRETE
  data: BRK_t input; T_tm output; tita_tm input; tita_l input; tita_hm input; vt_target input; vt_obs output; Kp_c parameter; Ki_c parameter; k_tita_c parameter; k_omega_c parameter; k_i_c parameter; Jt_eq parameter; g parameter; rhd parameter; ih parameter; rtd parameter; it parameter; Ts2 parameter; at_max parameter; vt_max parameter; Yt0 parameter; zitta parameter
function [T_tm, vt_obs] = nivel2_carro(BRK_t, tita_tm, tita_l, tita_hm, vt_target, Kp_c, Ki_c, k_tita_c, k_omega_c, k_i_c, Jt_eq, g, rhd, ih, rtd, it, Ts2, at_max, vt_max, Yt0, zitta)
%NIVEL2_CARRO  Nivel 2 control carro — pegar directamente en MATLAB Function block
%
%  Edit Data (Scope=Parameter, Type=double, Size=-1):
%    Kp_c, Ki_c, k_tita_c, k_omega_c, k_i_c,
%    Jt_eq, g, rhd, ih, rtd, it, Ts2, at_max, vt_max, Yt0, zitta
%#codegen

persistent T_out vt_out int_e prev_e theta_hat omega_hat x3 tita_prev rl_state T_prev;
if isempty(T_out)
    T_out     = 0;
    vt_out    = 0;
    int_e     = 0;
    prev_e    = 0;
    theta_hat = double(tita_tm);
    omega_hat = 0;
    x3        = 0;
    tita_prev = double(tita_tm);
    rl_state  = 0;
    T_prev    = 0;
end

% Output paso anterior — sin feedthrough directo → rompe bucle algebraico
T_tm   = T_out;
vt_obs = vt_out;

%% 1. Anti-sway
yh     = double(tita_hm) * (rhd / (2 * ih));
h      = max(Yt0 - yh, 0.5);
v_sway = double(tita_l) * 2 * zitta * sqrt(g * h);

%% 2. Corrección de referencia
vt_cmd   = double(vt_target) + v_sway;
vt_sat   = max(min(vt_cmd, vt_max), -vt_max);
delta    = vt_sat - rl_state;
rl_state = rl_state + max(min(delta, at_max * Ts2), -at_max * Ts2);
vt_ref   = rl_state;

%% 3. Observador de Luenberger
tita_delayed = tita_prev;
tita_prev    = double(tita_tm);

err_pos   = tita_delayed - theta_hat;
v_est     = omega_hat + k_tita_c * err_pos;
omega_dot = T_prev / Jt_eq + k_i_c * x3 + k_omega_c * err_pos;

theta_hat = theta_hat + Ts2 * v_est;
omega_hat = omega_hat + Ts2 * omega_dot;
x3        = x3        + Ts2 * err_pos;

vt_out = v_est * (rtd / it);

%% 4. PI trapezoidal con reset anti-windup
err = vt_ref - vt_out;
if ~double(BRK_t)
    int_e = 0;
else
    int_e = int_e + (Ts2 / 2) * (err + prev_e);
end
prev_e = err;

T_out  = Kp_c * err + Ki_c * int_e;
T_prev = T_out;

== matlab function planta_rots/Nivel 2/MATLAB Function1 ==
  data: BRK input; tita_hm input; T_hm output; m_cont input; vh_target input; vh_obs output; vh_max parameter; Ts2 parameter; ah_max parameter; Ms parameter; ih parameter; rhd parameter; g parameter; Jh_eq parameter; bh_eq parameter; k_i_h parameter; k_omega_h parameter; k_tita_h parameter; Ki_i parameter; Kp_i parameter
function [T_hm, vh_obs] = nivel2_izaje(BRK, tita_hm, m_cont, vh_target, vh_max, Ts2, ah_max, Ms, ih, rhd, g, Jh_eq, bh_eq, k_i_h, k_omega_h, k_tita_h, Ki_i, Kp_i)
%NIVEL2_IZAJE  Nivel 2 control izaje — pegar directamente en MATLAB Function block
%
%  Edit Data (Scope=Parameter, Type=double, Size=-1):
%    Kp_i, Ki_i, k_tita_h, k_omega_h, k_i_h,
%    Jh_eq, bh_eq, g, rhd, ih, Ms, Ts2, ah_max, vh_max
%#codegen

persistent T_out vh_out int_e prev_e theta_hat omega_hat x3 T_prev rl_state;
if isempty(T_out)
    T_out     = 0;
    vh_out    = 0;
    int_e     = 0;
    prev_e    = 0;
    theta_hat = double(tita_hm);
    omega_hat = 0;
    x3        = 0;
    T_prev    = 0;
    rl_state  = 0;
end

% Output paso anterior — sin feedthrough directo → rompe bucle algebraico
T_hm   = T_out;
vh_obs = vh_out;

%% 1. Modulación de referencia
vh_sat   = max(min(double(vh_target), vh_max), -vh_max);
delta    = vh_sat - rl_state;
rl_state = rl_state + max(min(delta, ah_max * Ts2), -ah_max * Ts2);
vh_ref   = rl_state;

%% 2. Observador de Luenberger
tita    = double(tita_hm);
err_pos = tita - theta_hat;

v_est     = omega_hat + k_tita_h * err_pos;
omega_dot = -(bh_eq / Jh_eq) * v_est + T_prev / Jh_eq ...
            + k_i_h * x3 + k_omega_h * err_pos;

theta_hat = theta_hat + Ts2 * v_est;
omega_hat = omega_hat + Ts2 * omega_dot;
x3        = x3        + Ts2 * err_pos;

vh_out = v_est * (rhd / (2 * ih));

%% 3. PI trapezoidal con reset anti-windup
err = vh_ref - vh_out;
if ~double(BRK)
    int_e = 0;
else
    int_e = int_e + (Ts2 / 2) * (err + prev_e);
end
prev_e = err;

m_total = Ms + double(m_cont);
T_out   = Kp_i * err + Ki_i * int_e + m_total * g * (rhd / (2 * ih));
T_prev  = T_out;
